simulink model "pvwindupfc11"  (R2016a)
settings: Solver=VariableStepAuto  StartTime=0.0  StopTime=0.5  RelTol=1e-3
undefined symbols (not defined in the file): BCMS11, c1, c2, c3, c4, c5, c6, Clink_3L, DiscIntNeverNeededParam, fdesignblkfcn, Fnom, gcbh, Ion, Ki_Ireg_3L, Ki_VDCreg_3L, Kp_Ireg_3L, Kp_VDCreg_3L, LimitL_Ireg_3L, LimitL_VDCreg_3L, LimitU_Ireg_3L, LimitU_VDCreg_3L, Lithium, LowerLimit, Pnom_3L, Pnom_dc_3L, PV11, Ts_Control, Ts_Power, Ts_PWM, UpperLimit, Vnom_dc_3L, Vnom_prim_3L, Vnom_sec_3L
libraries: powerlib x98, powerlib_extras x29, powerlib_meascontrol x20, fuzblock x2, simulink x1, electricdrivelib x1
(part 1 of 4)
settings Model: Creator=yaju  LastModifiedBy=yaju

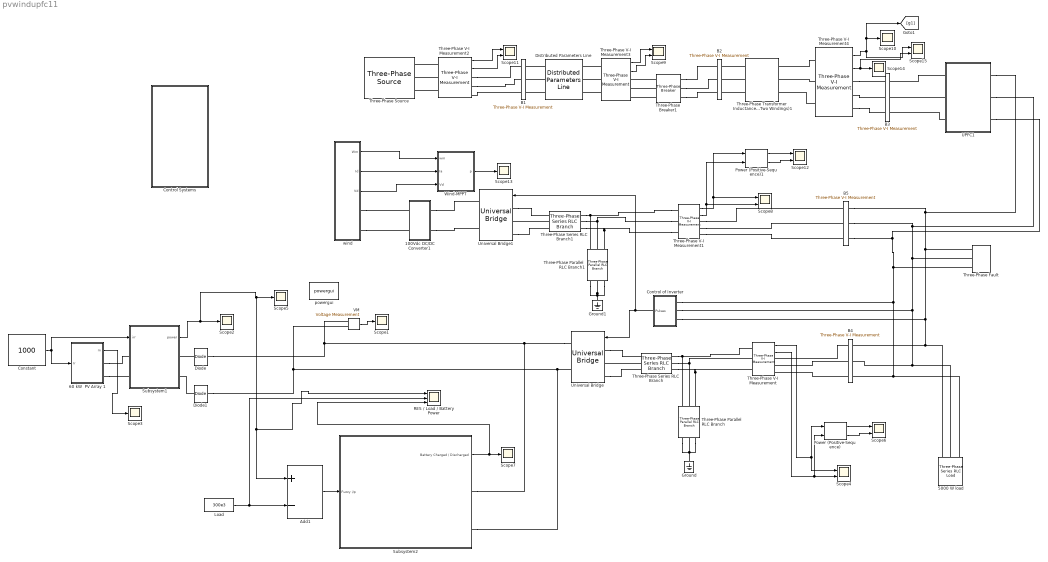
== system pvwindupfc11 ==
  100Vdc DC/DC Converter1 : Subsystem
  "5000 W load " : powerlib/Elements/Three-Phase Series RLC Load  LConnTagsString=A|B|C  Configuration=Y (grounded)  NominalVoltage=440  Vabc=[1e3 1e3 1e3]  Vabcp=[1e3 1e3 1e3]  NominalFrequency=50  UnbalancedPower=off  ActivePower=300e3  InductivePower=0  CapacitivePower=0  Pabc=[10e3 9e3 11e3]  QLabc=[100 90 110]  QCabc=[100 90 110]  Pabcp=[10e3 9e3 11e3]  QLabcp=[100 90 110]  QCabcp=[100 90 110]  Measurements=Branch voltages and currents  LoadType=constant PQ
  60 kW  PV Array 1 : Subsystem  mask(PV array){ModuleType=First Solar FS-272, Ncell=116, Nser=2, Npar=100, ModuleParameters=[ 94.5738  1.18103  70.558  1.01088 ], ModelParameters=[ 7.7692  1044.9  1.1116e-68  1.1898  2.3 ], Ts=10, PlotVI_module=off, PlotVI_array=off}
      mask prompts: ModuleType "Module type:"; Ncell "Number of cells per module"; Nser "Number of series-connected  modules per string"; Npar "Number of parallel strings"; ModuleParameters "Module specifications under STC  [  Voc, Isc, Vmp, Imp ]"; ModelParameters "Model parameters for 1 module [ Rs, Rp, Isat, Iph, Qd ]"; Ts "Sample time"; PlotVI_module "Display  I-V and  P-V characteritics of one module"; PlotVI_array "Display  I-V and  P-V characteritics of array"
      mask help:
      | Model a PV array
      |
      | PV array consists of Npar strings of modules connected in parallel, each string consisting of Nser modules connected in series.
      |
      | The four PV model parameters (photo-generated current Iph, diode saturation current Isat, parallel resistance Rp and  series resistance Rs) are adjuted to fit the following four module characteristics measured under standard test conditions (STC : irradiance 1000 W/m^2, cell temperature=25 deg. C) and assuming a given "diode quality factor" (Qd) for the semiconductor:
      |   Voc = open circuit voltage
      |   Isc = short-circuit current
      |   Vmp,Imp = voltage and current at maximum power point
      |
      | Select a 'Module type' and then press Apply to see module parameters.
      | Note: Module characteristics are extracted from NREL System Advisor Model.
      mask init:
      | BlockName=gcb;
      | 
      | % SolarModuleSpec_Definition_v2.m
      | %================================
      | %
      | Type=1;
      | SolarModuleSpec(Type).Desc= 'Kyocera KD135GX-LP';
      | SolarModuleSpec(Type).nCells= 36;              % Number of cells in series
      | SolarModuleSpec(Type).Pmp= 135.044;            % Maximum power (W)
      | SolarModuleSpec(Type).Vmp= 17.7;               % Maximum power voltage (V) 
      | SolarModuleSpec(Type).Imp= 7.62959;            % Maximum power current (A)
      | SolarModuleSpec(Type).Voc= 22.0999;            % Open circuit voltage (V)
      | SolarModuleSpec(Type).Isc= 8.36955;            % Short circuit current (A)
      | SolarModuleSpec(Type).TempC_Pmp= -6.445e-001;  % Maximum power temp. coefficient (W/deg.C)
      | SolarModuleSpec(Type).TempC_Vmp= -8.200e-002;  % Maximum power voltage temp. coefficient (V/deg.C)
      | SolarModuleSpec(Type).TempC_Imp= -1.068e-003;  % Maximum power current temp. coefficient (A/deg.C
      | SolarModuleSpec(Type).TempC_Voc= -8.000e-002;  % Open circuit voltage temp. coefficient (V/deg.C)
      | SolarModuleSpec(Type).TempC_Isc= 5.022e-003;   % Short circuit current temp. coefficient (A/deg.C)
      | SolarModuleSpec(Type).Rs= 0.10593;             % Series resistance of PV model (ohms)
      | SolarModuleSpec(Type).Rp= 142.84;              % Parallel resistance of PV model (ohms)
      | SolarModuleSpec(Type).Isat= 9.845e-07;         % Diode saturation current of PV model (A)
      | SolarModuleSpec(Type).Iph=  8.3758;            % Light-generated photo-current  of PV model (A)
      | SolarModuleSpec(Type).Qd= 1.5;                 % Diode quality factor of PV model
      | %-------------------------------------------------------------------------
      | %
      | Type=2;
      | SolarModuleSpec(Type).Desc= 'Kyocera KD205GX-LP';
      | SolarModuleSpec(Type).nCells= 54;              % Number of cells in series
      | SolarModuleSpec(Type).Pmp= 205.075;            % Maximum power (W)
      | SolarModuleSpec(Type).Vmp= 26.6;               % Maximum power voltage (V) 
      | SolarModuleSpec(Type).Imp= 7.70959;            % Maximum power current (A)
      | SolarModuleSpec(Type).Voc= 33.1999;            % Open circuit voltage (V)
      | SolarModuleSpec(Type).Isc= 8.35955;            % Short circuit current (A)
      | SolarModuleSpec(Type).TempC_Pmp= -9.770e-001;  % Maximum power temp. coefficient (W/deg.C)
      | SolarModuleSpec(Type).TempC_Vmp= -1.230e-001;  % Maximum power voltage temp. coefficient (V/deg.C)
      | SolarModuleSpec(Type).TempC_Imp= -1.079e-003;  % Maximum power current temp. coefficient (A/deg.C
      | SolarModuleSpec(Type).TempC_Voc= -1.200e-001;  % Open circuit voltage temp. coefficient (V/deg.C)
      | SolarModuleSpec(Type).TempC_Isc= 5.016e-003;   % Short circuit current temp. coefficient (A/deg.C)
      | SolarModuleSpec(Type).Rs= 0.15945;             % Series resistance of PV model (ohms)
      | SolarModuleSpec(Type).Rp= 1010.6;              % Parallel resistance of PV model (ohms)
      | SolarModuleSpec(Type).Isat=  9.7399e-07;       % Diode saturation current of PV model (A)
      | SolarModuleSpec(Type).Iph= 8.3642;             % Light-generated photo-current  of PV model (A)
      | SolarModuleSpec(Type).Qd= 1.5;                 % Diode quality factor of PV model
      | %-------------------------------------------------------------------------
      | %
      | Type=3;
      | SolarModuleSpec(Type).Desc= 'Mitsubishi PV-UD190MF5';
      | SolarModuleSpec(Type).nCells= 50;              % Number of cells in series
      | SolarModuleSpec(Type).Pmp= 190.503;            % Maximum power (W)
      | SolarModuleSpec(Type).Vmp= 24.6999;            % Maximum power voltage (V) 
      | SolarModuleSpec(Type).Imp= 7.71272;            % Maximum power current (A)
      | SolarModuleSpec(Type).Voc= 30.8006;            % Open circuit voltage (V)
      | SolarModuleSpec(Type).Isc= 8.23289;            % Short circuit current (A)
      | SolarModuleSpec(Type).TempC_Pmp= -8.597e-001;  % Maximum power temp. coefficient (W/deg.C)
      | SolarModuleSpec(Type).TempC_Vmp= -1.090e-001;  % Maximum power voltage temp. coefficient (V/deg.C)
      | SolarModuleSpec(Type).TempC_Imp= -7.713e-004;  % Maximum power current temp. coefficient (A/deg.C
      | SolarModuleSpec(Type).TempC_Voc= -1.050e-001;  % Open circuit voltage temp. coefficient (V/deg.C)
      | SolarModuleSpec(Type).TempC_Isc= 4.446e-003;   % Short circuit current temp. coefficient (A/deg.C)
      | SolarModuleSpec(Type).Rs= 0.20758;             % Series resistance of PV model (ohms)
      | SolarModuleSpec(Type).Rp= 975.6;               % Parallel resistance of PV model (ohms)
      | SolarModuleSpec(Type).Isat= 7.9676e-08;        % Diode saturation current of PV model (A)
      | SolarModuleSpec(Type).Iph= 8.2649;             % Light-generated photo-current  of PV model (A)
      | SolarModuleSpec(Type).Qd= 1.3;                 % Diode quality factor of PV model
      | %-------------------------------------------------------------------------
      | %
      | Type=4;
      | SolarModuleSpec(Type).Desc= 'Sanyo HIP-225HDE1';
      | SolarModuleSpec(Type).nCells= 60;              % Number of cells in series
      | SolarModuleSpec(Type).Pmp= 224.899;            % Maximum power (W)
      | SolarModuleSpec(Type).Vmp= 33.9;               % Maximum power voltage (V) 
      | SolarModuleSpec(Type).Imp= 6.63419;            % Maximum power current (A)
      | SolarModuleSpec(Type).Voc= 41.7984;            % Open circuit voltage (V)
      | SolarModuleSpec(Type).Isc= 7.13383;            % Short circuit current (A)
      | SolarModuleSpec(Type).TempC_Pmp= -6.925e-001;  % Maximum power temp. coefficient (W/deg.C)
      | SolarModuleSpec(Type).TempC_Vmp= -1.010e-001;  % Maximum power voltage temp. coefficient (V/deg.C)
      | SolarModuleSpec(Type).TempC_Imp= -6.634e-004;  % Maximum power current temp. coefficient (A/deg.C
      | SolarModuleSpec(Type).TempC_Voc= -1.050e-001;  % Open circuit voltage temp. coefficient (V/deg.C)
      | SolarModuleSpec(Type).TempC_Isc= 2.140e-003;   % Short circuit current temp. coefficient (A/deg.C)
      | SolarModuleSpec(Type).Rs=  0.20439;            % Series resistance of PV model (ohms)
      | SolarModuleSpec(Type).Rp= 1830.7;              % Parallel resistance of PV model (ohms)
      | SolarModuleSpec(Type).Isat=  3.0815e-07;       % Diode saturation current of PV model (A)
      | SolarModuleSpec(Type).Iph=  7.145;             % Light-generated photo-current  of PV model (A)
      | SolarModuleSpec(Type).Qd= 1.6;                 % Diode quality factor of PV model
      | %-------------------------------------------------------------------------
      | %
      | 
      | Type=5;
      | % NREL : 2007(E)
      | SolarModuleSpec(Type).Desc= 'SunPower SPR-305-WHT';
      | SolarModuleSpec(Type).nCells= 96;              % Number of cells in series
      | SolarModuleSpec(Type).Pmp= 305.2;              % Maximum power (W)
      | SolarModuleSpec(Type).Vmp= 54.70;              % Maximum power voltage (V) 
      | SolarModuleSpec(Type).Imp= 5.58;               % Maximum power current (A)
      | SolarModuleSpec(Type).Voc= 64.20;              % Open circuit voltage (V)
      | SolarModuleSpec(Type).Isc= 5.96;               % Short circuit current (A)
      | SolarModuleSpec(Type).TempC_Pmp= -1.154e+000;  % Maximum power temp. coefficient (W/deg.C)
      | SolarModuleSpec(Type).TempC_Vmp= -1.860e-001;  % Maximum power voltage temp. coefficient (V/deg.C)
      | SolarModuleSpec(Type).TempC_Imp= -2.120e-003;  % Maximum power current temp. coefficient (A/deg.C
      | SolarModuleSpec(Type).TempC_Voc= -1.770e-001;  % Open circuit voltage temp. coefficient (V/deg.C)
      | SolarModuleSpec(Type).TempC_Isc= 3.516e-003;   % Short circuit current temp. coefficient (A/deg.C)
      | SolarModuleSpec(Type).Rs= 0.037998;            % Series resistance of PV model (ohms)
      | SolarModuleSpec(Type).Rp= 993.51;              % Parallel resistance of PV model (ohms)
      | SolarModuleSpec(Type).Isat= 1.1753e-08;        % Diode saturation current of PV model (A)
      | SolarModuleSpec(Type).Iph= 5.9602;             % Light-generated photo-current  of PV model (A)
      | SolarModuleSpec(Type).Qd= 1.3;                 % Diode quality factor of PV model
      | %-------------------------------------------------------------------------
      | %
      | Type=6;
      | SolarModuleSpec(Type).Desc= 'Suntech STP270S-24_Vb';
      | SolarModuleSpec(Type).nCells= 72;              % Number of cells in series
      | SolarModuleSpec(Type).Pmp= 269.843;            % Maximum power (W)
      | SolarModuleSpec(Type).Vmp= 35;                 % Maximum power voltage (V) 
      | SolarModuleSpec(Type).Imp= 7.70979;            % Maximum power current (A)
      | SolarModuleSpec(Type).Voc= 44.4999;            % Open circuit voltage (V)
      | SolarModuleSpec(Type).Isc= 8.19978;            % Short circuit current (A)
      | SolarModuleSpec(Type).TempC_Pmp= -1.204e+000;  % Maximum power temp. coefficient (W/deg.C)
      | SolarModuleSpec(Type).TempC_Vmp= -1.567e-001;  % Maximum power voltage temp. coefficient (V/deg.C)
      | SolarModuleSpec(Type).TempC_Imp= 1.234e-004;   % Maximum power current temp. coefficient (A/deg.C
      | SolarModuleSpec(Type).TempC_Voc= -1.504e-001;  % Open circuit voltage temp. coefficient (V/deg.C)
      | SolarModuleSpec(Type).TempC_Isc= 4.969e-003;   % Short circuit current temp. coefficient (A/deg.C)
      | SolarModuleSpec(Type).Rs= 0.32025;             % Series resistance of PV model (ohms)
      | SolarModuleSpec(Type).Rp= 2562.3;              % Parallel resistance of PV model (ohms)
      | SolarModuleSpec(Type).Isat= 8.8992e-07;        % Diode saturation current of PV model (A)
      | SolarModuleSpec(Type).Iph= 8.2979;             % Light-generated photo-current  of PV model (A)
      | SolarModuleSpec(Type).Qd= 1.5;                 % Diode quality factor of PV model
      | % 
      | %-------------------------------------------------------------------------
      | %
      | Type=7;
      | SolarModuleSpec(Type).Desc= 'Canadian Solar CS5P-220M';
      | SolarModuleSpec(Type).nCells= 96;              % Number of cells in series
      | SolarModuleSpec(Type).Pmp= 219.72;             % Maximum power (W)
      | SolarModuleSpec(Type).Vmp= 48.3159;            % Maximum power voltage (V) 
      | SolarModuleSpec(Type).Imp= 4.54758;            % Maximum power current (A)
      | SolarModuleSpec(Type).Voc= 59.2618;            % Open circuit voltage (V)
      | SolarModuleSpec(Type).Isc= 5.09261;            % Short circuit current (A)
      | SolarModuleSpec(Type).TempC_Pmp= -1.031e+000;  % Maximum power temp. coefficient (W/deg.C)
      | SolarModuleSpec(Type).TempC_Vmp= -2.355e-001;  % Maximum power voltage temp. coefficient (V/deg.C)
      | SolarModuleSpec(Type).TempC_Imp= 8.231e-004;   % Maximum power current temp. coefficient (A/deg.C
      | SolarModuleSpec(Type).TempC_Voc= -2.170e-001;  % Open circuit voltage temp. coefficient (V/deg.C)
      | SolarModuleSpec(Type).TempC_Isc= 2.022e-003;   % Short circuit current temp. coefficient (A/deg.C)
      | SolarModuleSpec(Type).Rs= 0.24807;             % Series resistance of PV model (ohms)
      | SolarModuleSpec(Type).Rp= 235.76;              % Parallel resistance of PV model (ohms)
      | SolarModuleSpec(Type).Isat= 5.3103e-07;        % Diode saturation current of PV model (A)
      | SolarModuleSpec(Type).Iph= 5.098;              % Light-generated photo-current  of PV model (A)
      | SolarModuleSpec(Type).Qd= 1.5;                 % Diode quality factor of PV model
      | %-------------------------------------------------------------------------
      | %
      | Type=8;
      | SolarModuleSpec(Type).Desc= 'BP Solar SX3190';
      | SolarModuleSpec(Type).nCells= 50;              % Number of cells in series
      | SolarModuleSpec(Type).Pmp= 190.258;            % Maximum power (W)
      | SolarModuleSpec(Type).Vmp= 24.3003;            % Maximum power voltage (V) 
      | SolarModuleSpec(Type).Imp= 7.82945;            % Maximum power current (A)
      | SolarModuleSpec(Type).Voc= 30.6021;            % Open circuit voltage (V)
      | SolarModuleSpec(Type).Isc= 8.51029;            % Short circuit current (A)
      | SolarModuleSpec(Type).TempC_Pmp= -9.306e-001;  % Maximum power temp. coefficient (W/deg.C)
      | SolarModuleSpec(Type).TempC_Vmp= -1.140e-001;  % Maximum power voltage temp. coefficient (V/deg.C)
      | SolarModuleSpec(Type).TempC_Imp= -1.566e-003;  % Maximum power current temp. coefficient (A/deg.C
      | SolarModuleSpec(Type).TempC_Voc= -1.110e-001;  % Open circuit voltage temp. coefficient (V/deg.C)
      | SolarModuleSpec(Type).TempC_Isc= 5.532e-003;   % Short circuit current temp. coefficient (A/deg.C)
      | SolarModuleSpec(Type).Rs= 0.17514;             % Series resistance of PV model (ohms)
      | SolarModuleSpec(Type).Rp= 755.51;              % Parallel resistance of PV model (ohms)
      | SolarModuleSpec(Type).Isat= 1.0647e-06;       % Diode saturation current of PV model (A)
      | SolarModuleSpec(Type).Iph= 8.5158;             % Light-generated photo-current  of PV model (A)
      | SolarModuleSpec(Type).Qd= 1.5;                 % Diode quality factor of PV model
      | %-------------------------------------------------------------------------
      | %
      | Type=9;
      | SolarModuleSpec(Type).Desc= 'First Solar FS-272';
      | SolarModuleSpec(Type).nCells= 116;             % Number of cells in series
      | SolarModuleSpec(Type).Pmp= 71.326;             % Maximum power (W)
      | SolarModuleSpec(Type).Vmp= 70.558;             % Maximum power voltage (V) 
      | SolarModuleSpec(Type).Imp= 1.01088;            % Maximum power current (A)
      | SolarModuleSpec(Type).Voc= 94.5738;            % Open circuit voltage (V)
      | SolarModuleSpec(Type).Isc= 1.18103;            % Short circuit current (A)
      | SolarModuleSpec(Type).TempC_Pmp= -2.332e-001;  % Maximum power temp. coefficient (W/deg.C)
      | SolarModuleSpec(Type).TempC_Vmp= -2.060e-001;  % Maximum power voltage temp. coefficient (V/deg.C)
      | SolarModuleSpec(Type).TempC_Imp= -3.538e-004;  % Maximum power current temp. coefficient (A/deg.C
      | SolarModuleSpec(Type).TempC_Voc= -2.690e-001;  % Open circuit voltage temp. coefficient (V/deg.C)
      | SolarModuleSpec(Type).TempC_Isc= 5.433e-004;   % Short circuit current temp. coefficient (A/deg.C)
      | SolarModuleSpec(Type).Rs= 7.7692;              % Series resistance of PV model (ohms)
      | SolarModuleSpec(Type).Rp= 1044.9;              % Parallel resistance of PV model (ohms)
      | SolarModuleSpec(Type).Isat= 1.1116e-068;       % Diode saturation current of PV model (A)
      | SolarModuleSpec(Type).Iph= 1.1898;             % Light-generated photo-current  of PV model (A)
      | SolarModuleSpec(Type).Qd= 2.3;                 % Diode quality factor of PV model
      | %-------------------------------------------------------------------------
      | %
      | Type=10;
      | SolarModuleSpec(Type).Desc= 'SunPower 128-cell Module';
      | SolarModuleSpec(Type).nCells= 128;             % Number of cells in series
      | SolarModuleSpec(Type).Pmp= 400.048;            % Maximum power (W)
      | SolarModuleSpec(Type).Vmp= 72.8992;            % Maximum power voltage (V) 
      | SolarModuleSpec(Type).Imp= 5.48769;            % Maximum power current (A)
      | SolarModuleSpec(Type).Voc= 85.2983;            % Open circuit voltage (V)
      | SolarModuleSpec(Type).Isc= 5.8675;             % Short circuit current (A)
      | SolarModuleSpec(Type).TempC_Pmp= -1.638e+000;  % Maximum power temp. coefficient (W/deg.C)
      | SolarModuleSpec(Type).TempC_Vmp= -2.760e-001;  % Maximum power voltage temp. coefficient (V/deg.C)
      | SolarModuleSpec(Type).TempC_Imp= -1.690e-003;  % Maximum power current temp. coefficient (A/deg.C
      | SolarModuleSpec(Type).TempC_Voc= -2.664e-001;  % Open circuit voltage temp. coefficient (V/deg.C)
      | SolarModuleSpec(Type).TempC_Isc= 1.837e-003;   % Short circuit current temp. coefficient (A/deg.C)
      | SolarModuleSpec(Type).Rs= 0.12264;             % Series resistance of PV model (ohms)
      | SolarModuleSpec(Type).Rp= 859.93;              % Parallel resistance of PV model (ohms)
      | SolarModuleSpec(Type).Isat= 2.3385e-09;        % Diode saturation current of PV model (A)
      | SolarModuleSpec(Type).Iph= 5.8683;             % Light-generated photo-current  of PV model (A)
      | SolarModuleSpec(Type).Qd= 1.2;                 % Diode quality factor of PV model
      | %-------------------------------------------------------------------------
      | 
      | Type=strmatch(ModuleType,char(SolarModuleSpec.Desc));
      | 
      | k= 1.3806e-23; % Boltzman constant (J.K^-1)
      | q=1.6022e-19;  % electron charge  (C)
      | T=273+25;
      | 
      | nCells=SolarModuleSpec(Type).nCells;
      | Voc=SolarModuleSpec(Type).Voc;
      | Isc=SolarModuleSpec(Type).Isc;
      | Vm=SolarModuleSpec(Type).Vmp;
      | Im=SolarModuleSpec(Type).Imp;
      | 
      | set_param(BlockName,'Ncell',num2str(nCells));
      | str=sprintf('[ %g  %g  %g  %g ]',Voc,Isc,Vm,Im);
      | set_param(BlockName,'ModuleParameters',str);
      | 
      | Rs=SolarModuleSpec(Type).Rs;
      | Rp=SolarModuleSpec(Type).Rp; 
      | Isat=SolarModuleSpec(Type).Isat;
      | Iph=SolarModuleSpec(Type).Iph;            
      | Qd=SolarModuleSpec(Type).Qd;
      | 
      | VT=k*T/q*nCells*Qd;
      | 
      | str=sprintf('[ %g  %g  %g  %g  %g ]',Rs,Rp,Isat,Iph, Qd);
      | set_param(BlockName,'ModelParameters',str)
      | 
      | Iph_array=Iph*Npar;
      | Isat_array=Isat*Npar;
      | VT_array=VT*Nser;
      | Rs_array=Rs*Nser/Npar;
      | Rp_array=Rp*Nser/Npar;
      | %
      | %% Plot I-V & P-V characteristics of one module
      | %==============================================
      | if PlotVI_module | PlotVI_array
      |     assignin('base','Voc',Voc);
      |     assignin('base','Isc',Isc);
      |     assignin('base','Rs',Rs);
      |     assignin('base','Rp',Rp);
      |     assignin('base','Isat',Isat);
      |     assignin('base','VT',VT);
      |      
      |     if PlotVI_module, 
      |         F1=figure('Name','I-V and P-V characteristics of one module at 25 deg.C');
      |     end
      |     if PlotVI_array ,
      |         F2=figure('Name','I-V and P-V characteristics of array at 25 deg.C');  
      |     end
      |     load_system('PV_model_Param');
      |     
      |     for ksun=1:-0.25:0.25
      |         assignin('base','Iph',Iph*ksun)
      |         sim('PV_model_Param');
      |         n=find(I_PV>=0);
      |         I_PV=I_PV(n);
      |         V_PV=V_PV(n);
      |         P_PV=V_PV.*I_PV;
      |         
      |         if PlotVI_module
      |             figure(F1);
      |             subplot(211)
      |             if ksun==1
      |                 plot(V_PV,I_PV,'b',[0  Vm Voc], [Isc Im 0],'ro')
      |                 text(Voc/15,Isc*1.1,'1 kW/m^2')
      |                 hold on
      |                 grid
      |             else
      |                 plot(V_PV,I_PV,'--m')
      |                 text(Voc/15, Isc*(ksun+0.1) , sprintf('%g kW/m^2',ksun))
      |             end
      | 
      |             subplot(212) 
      |             if ksun==1
      |                 plot(V_PV,P_PV,'b',[0  Vm Voc], [0 Im*Vm 0],'ro')
      |                 text(Vm*1.02,Vm*Im,'1 kW/m^2')
      |                 hold on
      |                 grid
      |             else
      |                 n= find(P_PV==max(P_PV));
      |                 plot(V_PV,P_PV,'--m', V_PV(n) , P_PV(n),'mo')
      |                 text(Vm*1.02, Vm*Im*ksun, sprintf('%g kW/m^2',ksun))
      |             end
      |             subplot(211)
      |             ylabel('Current (A)')
      |             xlabel('Voltage (V)')
      |             title(sprintf('Module type: %s',SolarModuleSpec(Type).Desc))
      |             axis_xy=axis;
      |             axis_xy(4)=Isc*1.2;
      |             axis(axis_xy);
      |             
      |             subplot(212)
      |             ylabel('Power (W)')
      |             xlabel('Voltage (V)')
      |             axis_xy=axis;
      |             axis_xy(4)=Vm*Im*1.2;
      |             axis(axis_xy);
      |                   
      |             set_param(BlockName,'PlotVI_module', 'off')
      |         end
      |         
      |         if PlotVI_array
      |             figure(F2);
      |             subplot(211)
      |             if ksun==1
      |                 plot(V_PV*Nser,I_PV*Npar,'b',[0  Vm Voc]*Nser, [Isc Im 0]*Npar,'ro')
      |                 text(Voc/15*Nser,Isc*1.1*Npar,'1 kW/m^2')
      |                 hold on
      |                 grid
      |             else
      |                 plot(V_PV*Nser,I_PV*Npar,'--m')
      |                 text(Voc*Nser/15, Isc*Npar*(ksun+0.1) , sprintf('%g kW/m^2',ksun))
      |             end
      |            
      | 
      |             subplot(212)
      |             if ksun==1
      |                 plot(V_PV*Nser,P_PV*Nser*Npar,'b',[0  Vm Voc]*Nser, [0 Im*Vm 0]*Nser*Npar,'ro')
      |                 text(Vm*Nser*1.02,Vm*Im*Nser*Npar,'1 kW/m^2')
      |                 hold on
      |                 grid
      |             else
      |                 n= find(P_PV==max(P_PV));
      |                 plot(V_PV*Nser,P_PV*Nser*Npar,'--m', V_PV(n)*Nser , P_PV(n)*Nser*Npar,'mo')
      |                 text(Vm*Nser*1.02, Vm*Im*Nser*Npar*ksun, sprintf('%g kW/m^2',ksun))
      |             end 
      |             subplot(211)
      |             ylabel('Current (A)')
      |             xlabel('Voltage (V)')
      |             title(sprintf('Array type: %s; %d series modules; %d parallel strings',SolarModuleSpec(Type).Desc,Nser,Npar));
      |             axis_xy=axis;
      |             axis_xy(4)=Isc*Npar*1.2;
      |             axis(axis_xy);
      |             
      |             subplot(212)
      |             ylabel('Power (W)')
      |             xlabel('Voltage (V)')
      |             xis_xy=axis;
      |             axis_xy(4)=Vm*Im*Nser*Npar*1.2;
      |             axis(axis_xy);
      |             
      |             set_param(BlockName,'PlotVI_array', 'off')
      |         end
      |         
      |     end  
      | end
      mask TypeOptions ModuleType: BP Solar SX3190 | Canadian Solar CS5P-220M | First Solar FS-272 | Kyocera KD135GX-LP | Kyocera KD205GX-LP | Mitsubishi PV-UD190MF5 | Sanyo HIP-225HDE1 | SunPower SPR-305-WHT | SunPower SPR-400-WHT | Suntech STP270S-24_Vb
      mask Display: image(imread('panel.jpg'))
  Add1 : Sum  Inputs=+-
  B1 : powerlib/Measurements/Three-Phase V-I Measurement  VoltageMeasurement=phase-to-ground  SetLabelV=on  LabelV=Vabc_B1  Vpu=off  VpuLL=off  CurrentMeasurement=no  SetLabelI=off  LabelI=A1  Ipu=off  Pbase=100e6  Vbase=25e3  OutputType=Magnitude  PhasorSimulation=off  PSBequivalent=0
  B2 : powerlib/Measurements/Three-Phase V-I Measurement  VoltageMeasurement=phase-to-ground  SetLabelV=on  LabelV=Vabc_B2  Vpu=off  VpuLL=off  CurrentMeasurement=yes  SetLabelI=on  LabelI=A2  Ipu=off  Pbase=100e6  Vbase=440  OutputType=Magnitude  PhasorSimulation=off  PSBequivalent=0
  B3 : powerlib/Measurements/Three-Phase V-I Measurement  VoltageMeasurement=phase-to-ground  SetLabelV=on  LabelV=Vabc_B3  Vpu=off  VpuLL=off  CurrentMeasurement=yes  SetLabelI=on  LabelI=A1  Ipu=off  Pbase=100e6  Vbase=440  OutputType=Magnitude  PhasorSimulation=off  PSBequivalent=0
  B4 : powerlib/Measurements/Three-Phase V-I Measurement  VoltageMeasurement=phase-to-phase  SetLabelV=on  LabelV=VL  Vpu=off  VpuLL=off  CurrentMeasurement=yes  SetLabelI=on  LabelI=IL  Ipu=off  Pbase=100e6  Vbase=440  OutputType=Magnitude  PhasorSimulation=off  PSBequivalent=0
  B5 : powerlib/Measurements/Three-Phase V-I Measurement  VoltageMeasurement=phase-to-phase  SetLabelV=on  LabelV=Vw  Vpu=off  VpuLL=off  CurrentMeasurement=yes  SetLabelI=on  LabelI=Iw  Ipu=off  Pbase=100e6  Vbase=440  OutputType=Magnitude  PhasorSimulation=off  PSBequivalent=0
  Constant : Constant  Value=1000
  "Control Systems " : Subsystem
  Control of Inverter : Subsystem
  Diode : powerlib/Power Electronics/Diode  Ron=0.001  Lon=0  Vf=0.8  IC=0  UseSnubber=off  Rs=500  Cs=250e-9  Measurements=off
  Diode1 : powerlib/Power Electronics/Diode  Ron=0.001  Lon=0  Vf=0.8  IC=0  UseSnubber=off  Rs=500  Cs=250e-9  Measurements=off
  Distributed Parameters Line : powerlib/Elements/Distributed Parameters Line  Phases=3  Frequency=50  Resistance=[0.01273 0.3864]  Inductance="[0.9337e-3  4.1264e-3]"  Capacitance=[12.74e-9 7.751e-9]  Length=100  x1=[-0.000566 7.82030020709527e-11 21549.3598240347 -59884.1327335566;-0.000565 7.81696739622793e-11 21568.1719154532 -59877.3598474532;-0.000564 7.81363381385684e-11 21586.9818781784 -59870.5810516913;-0.000563 7.81029946031101e-11 21605.789710354 -59863.79634694;-0.000562 7.80696433591952e-11 21624.5954101236 -59857.0057338688;-0.000561 7.80362844101155e-11 21643.3989756313 -59850.209213148;-0.00056 7.80029177591632e-11 21662.200405021 -59843.4067854484;-0.000559 7.79695434096316e-11 21680.9996964373 -59836.5984514413;-0.000558 7.79361613648146e-11 21699.7968480248 -59829.7842117987;-0.000557 7.79027716280069e-11 21718.5918579281 -59822.9640671931;-0.000556 7.78693742025038e-11 21737.3847242924 -59816.1380182977;-0.000555 7.78359690916016e-11 21756.1754452628 -59809.3060657862;-0.000554 7.78025562985972e-11 21774.9640189847 -59802.4682103328;-0.000553 7.77691358267884e-11 21793.7504436039 -59795.6244526124;-0.000552 7.77357076794736e-11 21812.5347172661 -59788.7747933005;-0.000551 7.7702271859952e-11 21831.3168381175 -59781.919233073;-0.00055 7.76688283715237e-11 21850.0968043043 -59775.0577726067;-0.000549 7.76353772174893e-11 21868.874613973 -59768.1904125787;-0.000548 7.76019184011503e-11 21887.6502652703 -59761.3171536668;-0.000547 7.75684519258091e-11 21906.4237563431 -59754.4379965494;-0.000546 7.75349777947686e-11 21925.1950853385 -59747.5529419054;-0.000545 7.75014960113326e-11 21943.964250404 -59740.6619904143;-0.000544 7.74680065788056e-11 21962.731249687 -59733.7651427563;-0.000543 7.74345095004928e-11 21981.4960813354 -59726.8623996119;-0.000542 7.74010047797004e-11 22000.258743497 -59719.9537616626;-0.000541 7.7367492419735e-11 22019.0192343202 -59713.0392295902;-0.00054 7.73339724239043e-11 22037.7775519533 -59706.1188040771;-0.000539 7.73004447955165e-11 22056.533694545 -59699.1924858062;-0.000538 7.72669095378806e-11 22075.287660244 -59692.2602754613;-0.000537 7.72333666543065e-11 22094.0394471996 -59685.3221737265;-0.000536 7.71998161481047e-11 22112.7890535608 -59678.3781812866;-0.000535 7.71662580225865e-11 22131.5364774772 -59671.4282988269;-0.000534 7.7132692281064e-11 22150.2817170986 -59664.4725270333;-0.000533 7.709911892685e-11 22169.0247705748 -59657.5108665923;-0.000532 7.7065537963258e-11 22187.765636056 -59650.5433181911;-0.000531 7.70319493936023e-11 22206.5043116925 -59643.5698825173;-0.00053 7.6998353221198e-11 22225.2407956349 -59636.5905602591;-0.000529 7.69647494493609e-11 22243.975086034 -59629.6053521054;-0.000528 7.69311380814076e-11 22262.7071810408 -59622.6142587456;-0.000527 7.68975191206554e-11 22281.4370788064 -59615.6172808697;-0.000526 7.68638925704223e-11 22300.1647774824 -59608.6144191683;-0.000525 7.68302584340271e-11 22318.8902752203 -59601.6056743324;-0.000524 7.67966167147894e-11 22337.6135701721 -59594.591047054;-0.000523 7.67629674160295e-11 22356.3346604898 -59587.5705380252;-0.000522 7.67293105410685e-11 22375.0535443257 -59580.5441479389;-0.000521 7.66956460932282e-11 22393.7702198324 -59573.5118774887;-0.00052 7.6661974075831e-11 22412.4846851626 -59566.4737273686;-0.000519 7.66282944922003e-11 22431.1969384692 -59559.4296982732;-0.000518 7.65946073456601e-11 22449.9069779054 -59552.3797908978;-0.000517 7.65609126395353e-11 22468.6148016247 -59545.3240059381;-0.000516 7.65272103771514e-11 22487.3204077805 -59538.2623440906;-0.000515 7.64935005618345e-11 22506.0237945269 -59531.1948060522;-0.000514 7.64597831969119e-11 22524.7249600177 -59524.1213925203;-0.000513 7.64260582857112e-11 22543.4239024073 -59517.0421041933;-0.000512 7.63923258315609e-11 22562.1206198501 -59509.9569417696;-0.000511 7.63585858377903e-11 22580.815110501 -59502.8659059487;-0.00051 7.63248383077295e-11 22599.5073725147 -59495.7689974304;-0.000509 7.62910832447091e-11 22618.1974040464 -59488.666216915;-0.000508 7.62573206520607e-11 22636.8852032516 -59481.5575651037;-0.000507 7.62235505331164e-11 22655.5707682858 -59474.4430426981;-0.000506 7.61897728912093e-11 22674.2540973048 -59467.3226504002 ...(+32977 chars)]  x2=[-0.000566 2.88453530126769e-09 21660.2738172482 -60242.2219797169;-0.000565 2.8836398112331e-09 21679.198400246 -60235.4142312845;-0.000564 2.88274403659468e-09 21698.1208435926 -60228.600537855;-0.000563 2.88184797744082e-09 21717.0411454206 -60221.7809001009;-0.000562 2.88095163385998e-09 21735.9593038626 -60214.9553186954;-0.000561 2.8800550059406e-09 21754.8753170514 -60208.123794312;-0.00056 2.87915809377119e-09 21773.78918312 -60201.2863276251;-0.000559 2.87826089744028e-09 21792.7009002019 -60194.4429193094;-0.000558 2.87736341703639e-09 21811.6104664304 -60187.5935700403;-0.000557 2.87646565264813e-09 21830.5178799392 -60180.738280494;-0.000556 2.87556760436409e-09 21849.4231388623 -60173.8770513468;-0.000555 2.8746692722729e-09 21868.3262413338 -60167.0098832761;-0.000554 2.87377065646323e-09 21887.227185488 -60160.1367769596;-0.000553 2.87287175702376e-09 21906.1259694595 -60153.2577330757;-0.000552 2.87197257404322e-09 21925.022591383 -60146.3727523032;-0.000551 2.87107310761036e-09 21943.9170493936 -60139.4818353217;-0.00055 2.87017335781393e-09 21962.8093416264 -60132.5849828113;-0.000549 2.86927332474276e-09 21981.6994662168 -60125.6821954527;-0.000548 2.86837300848566e-09 22000.5874213004 -60118.7734739272;-0.000547 2.86747240913149e-09 22019.4732050131 -60111.8588189166;-0.000546 2.86657152676914e-09 22038.3568154909 -60104.9382311034;-0.000545 2.86567036148752e-09 22057.2382508702 -60098.0117111707;-0.000544 2.86476891337558e-09 22076.1175092872 -60091.0792598019;-0.000543 2.86386718252229e-09 22094.9945888789 -60084.1408776814;-0.000542 2.86296516901663e-09 22113.869487782 -60077.196565494;-0.000541 2.86206287294764e-09 22132.7422041336 -60070.2463239249;-0.00054 2.86116029440437e-09 22151.6127360712 -60063.2901536603;-0.000539 2.86025743347589e-09 22170.4810817323 -60056.3280553865;-0.000538 2.85935429025133e-09 22189.3472392546 -60049.3600297908;-0.000537 2.85845086481981e-09 22208.2112067761 -60042.3860775609;-0.000536 2.85754715727051e-09 22227.0729824351 -60035.406199385;-0.000535 2.8566431676926e-09 22245.9325643699 -60028.4203959521;-0.000534 2.85573889617532e-09 22264.7899507192 -60021.4286679517;-0.000533 2.85483434280791e-09 22283.6451396218 -60014.4310160737;-0.000532 2.85392950767964e-09 22302.4981292168 -60007.4274410088;-0.000531 2.85302439087982e-09 22321.3489176435 -60000.4179434483;-0.00053 2.85211899249779e-09 22340.1975030413 -59993.4025240839;-0.000529 2.8512133126229e-09 22359.0438835501 -59986.3811836081;-0.000528 2.85030735134453e-09 22377.8880573097 -59979.3539227139;-0.000527 2.84940110875211e-09 22396.7300224603 -59972.3207420947;-0.000526 2.84849458493507e-09 22415.5697771423 -59965.2816424447;-0.000525 2.84758777998289e-09 22434.4073194962 -59958.2366244588;-0.000524 2.84668069398506e-09 22453.2426476629 -59951.1856888321;-0.000523 2.84577332703111e-09 22472.0757597834 -59944.1288362606;-0.000522 2.84486567921059e-09 22490.906653999 -59937.0660674408;-0.000521 2.84395775061309e-09 22509.735328451 -59929.9973830697;-0.00052 2.84304954132821e-09 22528.5617812812 -59922.922783845;-0.000519 2.84214105144558e-09 22547.3860106315 -59915.842270465;-0.000518 2.84123228105489e-09 22566.2080146441 -59908.7558436283;-0.000517 2.84032323024581e-09 22585.0277914612 -59901.6635040346;-0.000516 2.83941389910806e-09 22603.8453392254 -59894.5652523836;-0.000515 2.8385042877314e-09 22622.6606560795 -59887.4610893761;-0.000514 2.8375943962056e-09 22641.4737401665 -59880.3510157131;-0.000513 2.83668422462045e-09 22660.2845896297 -59873.2350320963;-0.000512 2.8357737730658e-09 22679.0932026124 -59866.1131392283;-0.000511 2.8348630416315e-09 22697.8995772584 -59858.9853378117;-0.00051 2.83395203040743e-09 22716.7037117114 -59851.8516285501;-0.000509 2.83304073948351e-09 22735.5056041158 -59844.7120121476;-0.000508 2.83212916894968e-09 22754.3052526156 -59837.5664893088;-0.000507 2.83121731889591e-09 22773.1026553556 -59830.4150607389;-0.000506 2.83030518941219e-09 22791.8978104805 -59823.2577271438 ...(+32984 chars)]  x3=[-0.000566 2.49879098388694e-11 55.3357283970746 -229.0309972891;-0.000565 2.49923351041356e-11 55.4076778750351 -229.013601755378;-0.000564 2.49967579027572e-11 55.479621884477 -228.99618361892;-0.000563 2.50011782342977e-11 55.5515604182998 -228.978742881444;-0.000562 2.50055960983208e-11 55.6234934694034 -228.961279544673;-0.000561 2.50100114943905e-11 55.6954210306883 -228.943793610329;-0.00056 2.50144244220711e-11 55.7673430950555 -228.926285080139;-0.000559 2.50188348809269e-11 55.8392596554065 -228.90875395583;-0.000558 2.50232428705228e-11 55.9111707046436 -228.891200239133;-0.000557 2.50276483904236e-11 55.9830762356694 -228.87362393178;-0.000556 2.50320514401945e-11 56.0549762413871 -228.856025035506;-0.000555 2.50364520194009e-11 56.1268707147004 -228.838403552048;-0.000554 2.50408501276087e-11 56.1987596485136 -228.820759483145;-0.000553 2.50452457643836e-11 56.2706430357317 -228.803092830538;-0.000552 2.50496389292918e-11 56.3425208692599 -228.785403595972;-0.000551 2.50540296218998e-11 56.4143931420043 -228.767691781191;-0.00055 2.50584178417742e-11 56.4862598468712 -228.749957387945;-0.000549 2.5062803588482e-11 56.5581209767679 -228.732200417982;-0.000548 2.50671868615901e-11 56.6299765246018 -228.714420873057;-0.000547 2.50715676606662e-11 56.701826483281 -228.696618754923;-0.000546 2.50759459852777e-11 56.7736708457144 -228.678794065338;-0.000545 2.50803218349925e-11 56.8455096048111 -228.660946806061;-0.000544 2.50846952093788e-11 56.9173427534809 -228.643076978853;-0.000543 2.5089066108005e-11 56.9891702846341 -228.625184585478;-0.000542 2.50934345304396e-11 57.0609921911818 -228.607269627702;-0.000541 2.50978004762515e-11 57.1328084660354 -228.589332107293;-0.00054 2.51021639450098e-11 57.2046191021068 -228.571372026021;-0.000539 2.51065249362838e-11 57.2764240923086 -228.553389385659;-0.000538 2.51108834496432e-11 57.348223429554 -228.535384187983;-0.000537 2.51152394846578e-11 57.4200171067567 -228.517356434768;-0.000536 2.51195930408975e-11 57.4918051168309 -228.499306127794;-0.000535 2.51239441179329e-11 57.5635874526914 -228.481233268842;-0.000534 2.51282927153344e-11 57.6353641072536 -228.463137859698;-0.000533 2.51326388326728e-11 57.7071350734334 -228.445019902145;-0.000532 2.51369824695192e-11 57.7789003441473 -228.426879397973;-0.000531 2.51413236254448e-11 57.8506599123123 -228.408716348971;-0.00053 2.51456623000214e-11 57.9224137708462 -228.390530756933;-0.000529 2.51499984928205e-11 57.994161912667 -228.372322623654;-0.000528 2.51543322034143e-11 58.0659043306934 -228.35409195093;-0.000527 2.51586634313751e-11 58.1376410178449 -228.33583874056;-0.000526 2.51629921762753e-11 58.2093719670413 -228.317562994347;-0.000525 2.51673184376878e-11 58.2810971712029 -228.299264714093;-0.000524 2.51716422151855e-11 58.3528166232509 -228.280943901606;-0.000523 2.51759635083417e-11 58.4245303161067 -228.262600558693;-0.000522 2.518028231673e-11 58.4962382426926 -228.244234687164;-0.000521 2.5184598639924e-11 58.5679403959313 -228.225846288832;-0.00052 2.51889124774977e-11 58.6396367687459 -228.207435365512;-0.000519 2.51932238290255e-11 58.7113273540604 -228.189001919022;-0.000518 2.51975326940818e-11 58.7830121447993 -228.17054595118;-0.000517 2.52018390722413e-11 58.8546911338874 -228.152067463807;-0.000516 2.5206142963079e-11 58.9263643142504 -228.133566458729;-0.000515 2.52104443661701e-11 58.9980316788144 -228.11504293777;-0.000514 2.52147432810902e-11 59.0696932205061 -228.096496902759;-0.000513 2.52190397074148e-11 59.1413489322528 -228.077928355526;-0.000512 2.522333364472e-11 59.2129988069824 -228.059337297904;-0.000511 2.5227625092582e-11 59.2846428376233 -228.040723731728;-0.00051 2.52319140505772e-11 59.3562810171045 -228.022087658835;-0.000509 2.52362005182823e-11 59.4279133383557 -228.003429081064;-0.000508 2.52404844952742e-11 59.4995397943069 -227.984748000257;-0.000507 2.52447659811303e-11 59.571160377889 -227.966044418257;-0.000506 2.52490449754278e-11 59.6427750820333 -227.947318336911 ...(+32983 chars)]  x4=[-0.000566 -2.06337106483975e-11 79.7058223394571 -221.771405365322;-0.000565 -2.06391117100755e-11 79.7754899467736 -221.746354099163;-0.000564 -2.06445107347549e-11 79.8451496805649 -221.721280947516;-0.000563 -2.06499077219028e-11 79.9148015339558 -221.696185912856;-0.000562 -2.06553026709864e-11 79.984445500072 -221.671068997659;-0.000561 -2.06606955814735e-11 80.05408157204 -221.645930204406;-0.00056 -2.06660864528316e-11 80.1237097429868 -221.620769535576;-0.000559 -2.06714752845287e-11 80.1933300060406 -221.595586993652;-0.000558 -2.06768620760331e-11 80.26294235433 -221.570382581122;-0.000557 -2.06822468268129e-11 80.3325467809845 -221.545156300471;-0.000556 -2.06876295363369e-11 80.4021432791345 -221.51990815419;-0.000555 -2.06930102040736e-11 80.4717318419112 -221.49463814477;-0.000554 -2.06983888294922e-11 80.5413124624463 -221.469346274706;-0.000553 -2.07037654120616e-11 80.6108851338725 -221.444032546494;-0.000552 -2.07091399512514e-11 80.6804498493234 -221.418696962632;-0.000551 -2.07145124465309e-11 80.7500066019331 -221.393339525621;-0.00055 -2.07198828973701e-11 80.8195553848366 -221.367960237963;-0.000549 -2.07252513032388e-11 80.8890961911699 -221.342559102163;-0.000548 -2.07306176636072e-11 80.9586290140694 -221.317136120729;-0.000547 -2.07359819779456e-11 81.0281538466725 -221.291691296169;-0.000546 -2.07413442457247e-11 81.0976706821175 -221.266224630995;-0.000545 -2.07467044664152e-11 81.1671795135432 -221.24073612772;-0.000544 -2.0752062639488e-11 81.2366803340895 -221.215225788859;-0.000543 -2.07574187644144e-11 81.3061731368969 -221.189693616931;-0.000542 -2.07627728406656e-11 81.3756579151068 -221.164139614456;-0.000541 -2.07681248677134e-11 81.4451346618611 -221.138563783955;-0.00054 -2.07734748450293e-11 81.514603370303 -221.112966127953;-0.000539 -2.07788227720856e-11 81.584064033576 -221.087346648976;-0.000538 -2.07841686483542e-11 81.6535166448247 -221.061705349552;-0.000537 -2.07895124733076e-11 81.7229611971944 -221.036042232213;-0.000536 -2.07948542464184e-11 81.7923976838312 -221.010357299492;-0.000535 -2.08001939671594e-11 81.861826097882 -220.984650553922;-0.000534 -2.08055316350035e-11 81.9312464324945 -220.958921998042;-0.000533 -2.0810867249424e-11 82.0006586808171 -220.93317163439;-0.000532 -2.08162008098942e-11 82.0700628359992 -220.907399465509;-0.000531 -2.08215323158878e-11 82.1394588911908 -220.881605493942;-0.00053 -2.08268617668785e-11 82.2088468395428 -220.855789722234;-0.000529 -2.08321891623403e-11 82.2782266742069 -220.829952152933;-0.000528 -2.08375145017476e-11 82.3475983883356 -220.80409278859;-0.000527 -2.08428377845746e-11 82.4169619750822 -220.778211631757;-0.000526 -2.08481590102959e-11 82.4863174276007 -220.752308684987;-0.000525 -2.08534781783865e-11 82.5556647390461 -220.726383950839;-0.000524 -2.08587952883213e-11 82.6250039025741 -220.700437431869;-0.000523 -2.08641103395755e-11 82.6943349113411 -220.67446913064;-0.000522 -2.08694233316246e-11 82.7636577585044 -220.648479049714;-0.000521 -2.08747342639442e-11 82.8329724372222 -220.622467191656;-0.00052 -2.08800431360101e-11 82.9022789406534 -220.596433559033;-0.000519 -2.08853499472984e-11 82.9715772619576 -220.570378154415;-0.000518 -2.08906546972853e-11 83.0408673942955 -220.544300980374;-0.000517 -2.08959573854472e-11 83.1101493308284 -220.518202039483;-0.000516 -2.09012580112608e-11 83.1794230647184 -220.492081334318;-0.000515 -2.09065565742029e-11 83.2486885891284 -220.465938867457;-0.000514 -2.09118530737506e-11 83.3179458972222 -220.43977464148;-0.000513 -2.09171475093812e-11 83.3871949821645 -220.413588658969;-0.000512 -2.09224398805721e-11 83.4564358371206 -220.38738092251;-0.000511 -2.09277301868009e-11 83.5256684552567 -220.361151434688;-0.00051 -2.09330184275456e-11 83.5948928297398 -220.334900198092;-0.000509 -2.09383046022842e-11 83.6641089537378 -220.308627215313;-0.000508 -2.0943588710495e-11 83.7333168204192 -220.282332488945;-0.000507 -2.09488707516564e-11 83.8025164229536 -220.256016021582 ...(+33539 chars)]  x5=0.000565541566995743  V1=[6.391e-28 1.447e-27 1.033e-27 3.131e-10 6.364e+04 6.364e+04;0 0 0 314.2 314.2 314.2;1.571 1.571 1.571 -0.9014 0.4149 -1.156]  V2=[2.83e-26 3.509e-27 2.506e-27 7.829e-09 6.402e+04 6.402e+04;0 0 0 314.2 314.2 314.2;1.571 1.571 1.571 -1.069 0.4146 -1.156]  I1=[6.979e-28 1.622e-27 1.158e-27 5.456e-11 235.6 235.6;0 0 0 314.2 314.2 314.2;1.571 1.571 1.571 -2.349 0.3065 -1.264]  I2=[6.598e-28 1.603e-27 1.145e-27 5.164e-11 235.7 235.7;0 0 0 314.2 314.2 314.2;4.712 4.712 4.712 0.5907 0.4145 -1.156]  nHarmo=2  Measurements=None
  Ground : powerlib/Elements/Ground  LConnTagsString=a
  Ground1 : powerlib/Elements/Ground  LConnTagsString=a
  Load : Constant  Value=300e3
  Power (Positive-Sequence) : powerlib_meascontrol/Measurements/Power (Positive-Sequence)  Freq=60  Vinit=[0, 0]  Iinit=[0, 0]  Ts=0
  Power (Positive-Sequence)1 : powerlib_meascontrol/Measurements/Power (Positive-Sequence)  Freq=60  Vinit=[0, 0]  Iinit=[0, 0]  Ts=0
  "RES / Load / Battery Power " : Scope  NumInputPorts=3
  Scope{1..3,5,7,10,13..14} (8 alike) : Scope
  Scope{4,6,8..9,11..12,15} (7 alike) : Scope  NumInputPorts=2
  Subsystem1 : Subsystem
  Subsystem2 : Subsystem
  Three-Phase Parallel RLC Branch : powerlib/Elements/Three-Phase Parallel RLC Branch  LConnTagsString=A|B|C  RConnTagsString=A|B|C  BranchType=C  Resistance=1  Inductance=1e-3  Capacitance=13.5e-4  Measurements=None
  Three-Phase Parallel RLC Branch1 : powerlib/Elements/Three-Phase Parallel RLC Branch  LConnTagsString=A|B|C  RConnTagsString=A|B|C  BranchType=C  Resistance=1  Inductance=1e-3  Capacitance=13.5e-4  Measurements=None
  Three-Phase Series RLC Branch : powerlib/Elements/Three-Phase Series RLC Branch  LConnTagsString=A|B|C  RConnTagsString=A|B|C  BranchType=RL  Resistance=2  Inductance=1e-2  Capacitance=15.5e-5  Measurements=None
  Three-Phase Series RLC Branch1 : powerlib/Elements/Three-Phase Series RLC Branch  LConnTagsString=A|B|C  RConnTagsString=A|B|C  BranchType=RL  Resistance=2  Inductance=1e-2  Capacitance=15.5e-5  Measurements=None
  Three-Phase V-I Measurement : powerlib/Measurements/Three-Phase V-I Measurement  VoltageMeasurement=phase-to-phase  SetLabelV=off  LabelV=Vabc  Vpu=off  VpuLL=off  CurrentMeasurement=yes  SetLabelI=off  LabelI=Iabc  Ipu=off  Pbase=100e6  Vbase=500e3  OutputType=Complex  PhasorSimulation=off  PSBequivalent=0
  Three-Phase V-I Measurement1 : powerlib/Measurements/Three-Phase V-I Measurement  VoltageMeasurement=phase-to-phase  SetLabelV=off  LabelV=Vabc  Vpu=off  VpuLL=off  CurrentMeasurement=yes  SetLabelI=off  LabelI=Iabc  Ipu=off  Pbase=100e6  Vbase=500e3  OutputType=Complex  PhasorSimulation=off  PSBequivalent=0
  Three-Phase V-I Measurement2 : powerlib/Measurements/Three-Phase V-I Measurement  VoltageMeasurement=phase-to-ground  SetLabelV=off  LabelV=Vabc  Vpu=off  VpuLL=off  CurrentMeasurement=yes  SetLabelI=off  LabelI=Iabc  Ipu=off  Pbase=100e6  Vbase=500e3  OutputType=Complex  PhasorSimulation=off  PSBequivalent=0
  Three-Phase V-I Measurement3 : powerlib/Measurements/Three-Phase V-I Measurement  VoltageMeasurement=phase-to-ground  SetLabelV=off  LabelV=Vabc  Vpu=off  VpuLL=off  CurrentMeasurement=yes  SetLabelI=off  LabelI=Iabc  Ipu=off  Pbase=100e6  Vbase=500e3  OutputType=Complex  PhasorSimulation=off  PSBequivalent=0
  Three-Phase V-I Measurement4 : powerlib/Measurements/Three-Phase V-I Measurement  VoltageMeasurement=phase-to-phase  SetLabelV=off  LabelV=Vabc  Vpu=off  VpuLL=off  CurrentMeasurement=yes  SetLabelI=off  LabelI=Iabc  Ipu=off  Pbase=100e6  Vbase=500e3  OutputType=Complex  PhasorSimulation=off  PSBequivalent=0
  Three-Phase Breaker1 : powerlib/Elements/Three-Phase Breaker  InitialState=closed  SwitchA=off  SwitchB=off  SwitchC=off  SwitchTimes="[1/50  20/50]"  External=off  BreakerResistance=0.001  SnubberResistance=1e6  SnubberCapacitance=inf  Measurements=None
  Three-Phase Fault : powerlib/Elements/Three-Phase Fault  InitialStates=0  FaultA=on  FaultB=off  FaultC=off  GroundFault=on  SwitchTimes=[0.1 0.3]  External=off  SwitchStatus=NaN  FaultResistance=0.001  GroundResistance=0.01  SnubberResistance=1e6  SnubberCapacitance=inf  Measurements=None
  Three-Phase Source : powerlib/Electrical Sources/Three-Phase Source  InternalConnection=Yg  VoltagePhases=off  Voltage=63510.4  PhaseAngle=0  Voltage_phases=[25e3 25e3 25e3]/sqrt(3)  PhaseAngles_phases=[0 -120 +120]  Frequency=50  NonIdealSource=on  SpecifyImpedance=off  Resistance=0.8929  Inductance=16.58e-3  ShortCircuitLevel=100e6  BaseVoltage=63510.4  XRratio=7  BusType=swing  Pref=0  Qref=0  Prefabc=[10e3, 10e3, 10e3]  Qrefabc=[0, 0, 0]  Qmin=-inf  Qmax=inf
  Three-Phase Transformer Inductance Matrix Type (Two Windings)1 : powerlib/Elements/Three-Phase Transformer Inductance Matrix Type (Two Windings)  CoreType=Three-limb or five-limb core  Winding1Connection=Yg  Winding2Connection=Yg  AutoTransformer=off  Measurements=None  NominalPower=[100e3 50]  VLLnom="[63510.4  254.4]"  WindingResistances=[0.01 0.01]  NoLoadIexcPos=2  NoLoadPlossPos=1000  ShortCircuitReactancePos=0.06  ShortCircuitReactancePosAuto=0.06  NoLoadIexcZero=100  NoLoadPlossZero=1500  ShortCircuitReactanceZero=0.03  ShortCircuitReactanceZeroAuto=0.03
  UPFC1 : Subsystem
  Universal Bridge : powerlib/Power Electronics/Universal Bridge  Arms=3  SnubberResistance=1e5  SnubberCapacitance=inf  Device=MOSFET / Diodes  Ron=1e-3  Lon=0  ForwardVoltages="[  0  0  ]"  ForwardVoltage=0  GTOparameters=[ 10e-6 , 20e-6 ]  IGBTparameters=[ 1e-6 , 2e-6 ]  Measurements=None  Measurements_2=None  converterType=Rectifier
  Universal Bridge1 : powerlib/Power Electronics/Universal Bridge  Arms=3  SnubberResistance=1e5  SnubberCapacitance=inf  Device=MOSFET / Diodes  Ron=1e-3  Lon=0  ForwardVoltages="[  0  0  ]"  ForwardVoltage=0  GTOparameters=[ 10e-6 , 20e-6 ]  IGBTparameters=[ 1e-6 , 2e-6 ]  Measurements=None  Measurements_2=None  converterType=Rectifier
  VM : powerlib/Measurements/Voltage Measurement  PhasorSimulation=off  OutputType=Complex  PSBequivalent=0
  Wind-MPPT : Subsystem
  powergui : powerlib/powergui  Priority=1  SimulationMode=Discrete  SolverType=Tustin  SampleTime=1e-6  frequency=60  SPID=off  DisableSnubberDevices=off  DisableRonSwitches=off  DisableVfSwitches=off  SwTol=0  DisplayEquations=off  Interpol=off  ExternalGateDelay=off  methode=off  Ts=0  FunctionMessages=off  echomessages=off  HookPort=off  EnableUseOfTLC=off  x0status=blocks  frequencyindice=0  Pbase=100e6  ErrMax=1e-4  Iterations=50  UnitsV=kV  UnitsW=MW  buscounter=0  RestoreLinks=warning  ResistiveCurrentMeasurement=off  Frange=[0:2:500]  Ylog=off  Xlog=on  ShowGrid=off  save=off  variable=ZData  structure=gv1  ZoomFFT=off  StartTime=0.0  cycles=3  DisplayStyle=1  fundamental=50  FreqAxis=off  MaxFrequency=1000  frequencyindicesteady=1  RmsSteady=1  display=off
  wind : Subsystem
  wires:
  Constant/1 -> 60 kW  PV Array 1/1(Ir), Subsystem1/1(irr)
  60 kW  PV Array 1/1(m) -> Scope3/1
  Subsystem1/1("power ") -> Add1/1, "RES / Load / Battery Power "/1, Scope5/1, Scope2/1
  Control of Inverter/1(Pulses) -> Universal Bridge1/1, Universal Bridge/1
  VM/1 -> Scope1/1
  Add1/1 -> Subsystem2/1(Fuzzy i/p)
  Subsystem2/1("Battery Charged / Discharged ") -> "RES / Load / Battery Power "/3, Scope7/1
  Load/1 -> "RES / Load / Battery Power "/2, Add1/2
  Three-Phase V-I Measurement/1 -> Scope4/1, Power (Positive-Sequence)/1
  Three-Phase V-I Measurement/2 -> Scope4/2, Power (Positive-Sequence)/2
  Power (Positive-Sequence)/1 -> Scope6/1
  Power (Positive-Sequence)/2 -> Scope6/2
  Three-Phase V-I Measurement3/1 -> Scope9/1
  Three-Phase V-I Measurement3/2 -> Scope9/2
  Three-Phase V-I Measurement2/1 -> Scope11/1
  Three-Phase V-I Measurement2/2 -> Scope11/2
  Three-Phase V-I Measurement4/1 -> [g1], Scope10/1, Scope15/1
  Power (Positive-Sequence)1/1 -> Scope12/1
  Power (Positive-Sequence)1/2 -> Scope12/2
  Three-Phase V-I Measurement1/1 -> Scope8/1, Power (Positive-Sequence)1/1
  Three-Phase V-I Measurement1/2 -> Scope8/2, Power (Positive-Sequence)1/2
  wind/3(Vd) -> Wind-MPPT/3(Vd)
  wind/2(Id) -> Wind-MPPT/2(Ia)
  wind/1(Wm) -> Wind-MPPT/1(wm)
  Wind-MPPT/1(p) -> Scope13/1
  Three-Phase V-I Measurement4/2 -> Scope15/2, Scope14/1
  connections:
  Diode1/RConn1 -- VM/LConn2 -- Subsystem2/RConn2 -- Universal Bridge/RConn2
  Universal Bridge/RConn1 -- Subsystem2/RConn1 -- Diode/RConn1 -- VM/LConn1
  Three-Phase Parallel RLC Branch/LConn1 -- Three-Phase Series RLC Branch/RConn1 -- Three-Phase V-I Measurement/LConn1
  Three-Phase Series RLC Branch/RConn2 -- Three-Phase Parallel RLC Branch/LConn2 -- Three-Phase V-I Measurement/LConn2
  Three-Phase Series RLC Branch/RConn3 -- Three-Phase Parallel RLC Branch/LConn3 -- Three-Phase V-I Measurement/LConn3
  Three-Phase Parallel RLC Branch/RConn1 -- Three-Phase Parallel RLC Branch/RConn2 -- Three-Phase Parallel RLC Branch/RConn3 -- Ground/LConn1
  B4/LConn1 -- "5000 W load "/LConn1 -- UPFC1/RConn1 -- B5/LConn1 -- Three-Phase Fault/LConn1 -- Control of Inverter/LConn3
  B4/LConn2 -- "5000 W load "/LConn2 -- UPFC1/RConn2 -- B5/LConn2 -- Three-Phase Fault/LConn2 -- Control of Inverter/LConn2
  B4/LConn3 -- "5000 W load "/LConn3 -- B5/LConn3 -- UPFC1/RConn3 -- Three-Phase Fault/LConn3 -- Control of Inverter/LConn1
  Three-Phase V-I Measurement1/LConn1 -- Three-Phase Parallel RLC Branch1/LConn1 -- Three-Phase Series RLC Branch1/RConn1
  Three-Phase V-I Measurement1/LConn2 -- Three-Phase Series RLC Branch1/RConn2 -- Three-Phase Parallel RLC Branch1/LConn2
  Three-Phase V-I Measurement1/LConn3 -- Three-Phase Series RLC Branch1/RConn3 -- Three-Phase Parallel RLC Branch1/LConn3
  Three-Phase Parallel RLC Branch1/RConn3 -- Three-Phase Parallel RLC Branch1/RConn1 -- Ground1/LConn1 -- Three-Phase Parallel RLC Branch1/RConn2
  Three-Phase Series RLC Branch/LConn2 -- Universal Bridge/LConn2
  B4/RConn3 -- Three-Phase V-I Measurement/RConn3
  B4/RConn2 -- Three-Phase V-I Measurement/RConn2
  Three-Phase V-I Measurement4/LConn3 -- Three-Phase Transformer Inductance Matrix Type (Two Windings)1/RConn3
  Three-Phase V-I Measurement2/LConn2 -- Three-Phase Source/RConn2
  Three-Phase Transformer Inductance Matrix Type (Two Windings)1/LConn2 -- B2/LConn2
  Three-Phase Transformer Inductance Matrix Type (Two Windings)1/LConn1 -- B2/LConn1
  Three-Phase V-I Measurement3/LConn2 -- Distributed Parameters Line/RConn2
  Three-Phase V-I Measurement4/RConn3 -- B3/RConn3
  Three-Phase Breaker1/LConn1 -- B2/RConn1
  100Vdc DC/DC Converter1/RConn2 -- Universal Bridge1/RConn2
  Distributed Parameters Line/LConn3 -- B1/LConn3
  100Vdc DC/DC Converter1/RConn1 -- Universal Bridge1/RConn1
  wind/RConn2 -- 100Vdc DC/DC Converter1/LConn2
  Three-Phase V-I Measurement2/LConn1 -- Three-Phase Source/RConn1
  Three-Phase Breaker1/RConn2 -- Three-Phase V-I Measurement3/RConn2
  Three-Phase Series RLC Branch1/LConn2 -- Universal Bridge1/LConn2
  Three-Phase Breaker1/LConn3 -- B2/RConn3
  Three-Phase V-I Measurement1/RConn3 -- B5/RConn3
  Distributed Parameters Line/LConn1 -- B1/LConn1
  Three-Phase V-I Measurement4/RConn1 -- B3/RConn1
  wind/RConn1 -- 100Vdc DC/DC Converter1/LConn1
  Three-Phase V-I Measurement1/RConn1 -- B5/RConn1
  Three-Phase V-I Measurement1/RConn2 -- B5/RConn2
  Three-Phase V-I Measurement3/LConn1 -- Distributed Parameters Line/RConn1
  B4/RConn1 -- Three-Phase V-I Measurement/RConn1
  60 kW  PV Array 1/RConn1 -- Subsystem1/LConn1
  Universal Bridge/LConn1 -- Three-Phase Series RLC Branch/LConn1
  Diode/LConn1 -- Subsystem1/RConn1
  60 kW  PV Array 1/RConn2 -- Subsystem1/LConn2
  Diode1/LConn1 -- Subsystem1/RConn2
  Three-Phase V-I Measurement2/RConn3 -- B1/RConn3
  Three-Phase V-I Measurement2/RConn2 -- B1/RConn2
  Three-Phase V-I Measurement3/LConn3 -- Distributed Parameters Line/RConn3
  Three-Phase V-I Measurement4/LConn2 -- Three-Phase Transformer Inductance Matrix Type (Two Windings)1/RConn2
  Three-Phase V-I Measurement2/RConn1 -- B1/RConn1
  Three-Phase Breaker1/RConn3 -- Three-Phase V-I Measurement3/RConn3
  Universal Bridge1/LConn3 -- Three-Phase Series RLC Branch1/LConn3
  Three-Phase Breaker1/RConn1 -- Three-Phase V-I Measurement3/RConn1
  Universal Bridge/LConn3 -- Three-Phase Series RLC Branch/LConn3
  Three-Phase Breaker1/LConn2 -- B2/RConn2
  Three-Phase V-I Measurement4/LConn1 -- Three-Phase Transformer Inductance Matrix Type (Two Windings)1/RConn1
  Distributed Parameters Line/LConn2 -- B1/LConn2
  Three-Phase V-I Measurement4/RConn2 -- B3/RConn2
  Universal Bridge1/LConn1 -- Three-Phase Series RLC Branch1/LConn1
  Three-Phase Transformer Inductance Matrix Type (Two Windings)1/LConn3 -- B2/LConn3
  Three-Phase V-I Measurement2/LConn3 -- Three-Phase Source/RConn3
  UPFC1/LConn1 -- B3/LConn1
  UPFC1/LConn2 -- B3/LConn2
  UPFC1/LConn3 -- B3/LConn3
